simulink model "base_for_gendata"  (R2025a)
settings: Solver=VariableStepAuto  StartTime=0.0  StopTime=inf  RelTol=1e-3
undefined symbols (not defined in the file): Sim3dSensor
libraries: aerolibsim3d x2, sim3dcameralib x1, sl3dlib x1, sim3dphyssensorlib x1, sim3dlib x1, visionsinks x1
settings Model: Creator=Алексей  LastModifiedBy=Алексей

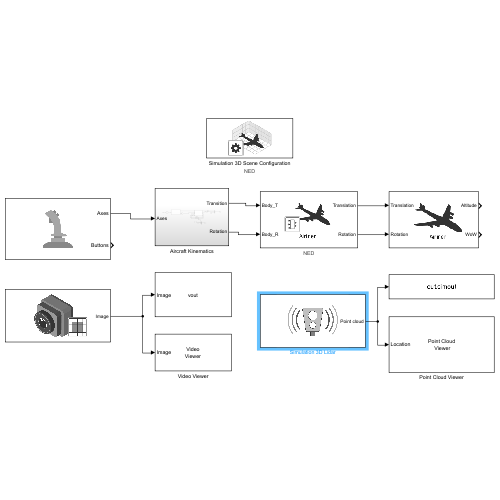
[thumbnail: Simulink's stored preview of the top-level diagram]
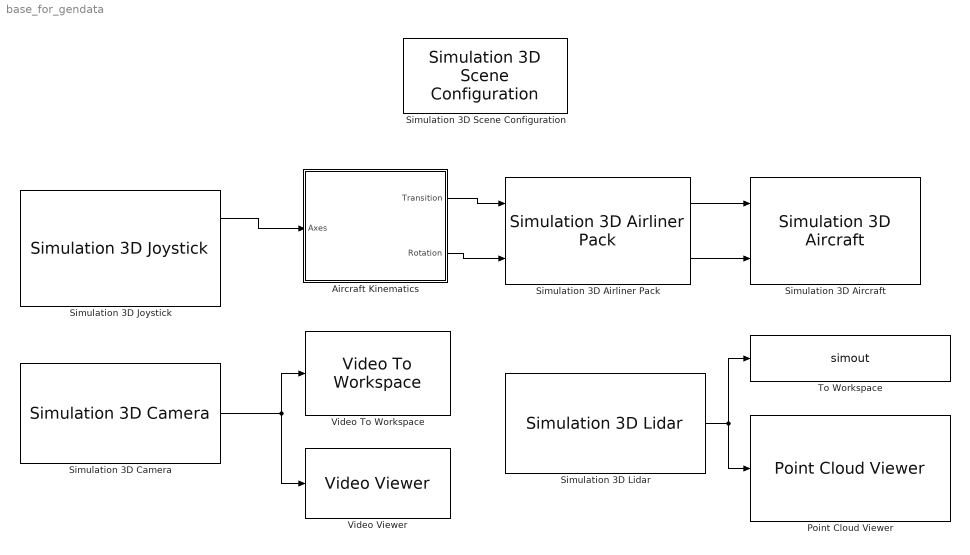
== system base_for_gendata ==
  Aircraft Kinematics : Subsystem
  Point Cloud Viewer : PointCloudViewer  FigPos=[2599 988 1022 472]  FigSettingsValue=[-1 138.910766601562 -120.239807128906 120.152908325195 -3.03508996963501 1 1]
  Simulation 3D Aircraft : aerolibsim3d/Simulation 3D Aircraft  Priority=-1  Mesh=Airliner  MeshPath=/MathWorksAerospaceContent/Vehicles/Aircraft/Custom/Mesh/SK_HL20.SK_HL20  MeshPathAT=/MathWorksAerospaceContent/Vehicles/Aircraft/AirTransport/Mesh/SK_AirTransport.SK_AirTransport  MeshPathGA=/MathWorksAerospaceContent/Vehicles/Aircraft/GeneralAviation/Mesh/SK_GeneralAviation.SK_GeneralAviation  AircraftColor=Red  ActorName=SimulinkVehicle1  Translation=repmat([0, 0, -3.030] + [0, 0, -0.01], 12, 1)  Rotation=repmat([0, -0.00021, 0], 12, 1)  ScaleInputPort=Dialog  Scale=[1 1 1]  InitialScale=[1 1 1]  IsGHSensorEnabled=on  AreGHRaysVisible=off  IsOutputReshapeEnabled=off  GHRayLength=1524  GHBodyOffset=0.90  GHFrontTireRadius=0.21  GHLeftTireRadius=0.21  GHRightTireRadius=0.21  WoWSensorTolerance=0.05  LightsConfig=Automatic lights  LandingLightIntensity=300000  LandingLightConeAngle=15  CustomLeftLandingLightLocation=[0 0 0]  CustomLeftLandingLightOrientation=[0 0 0]  CustomRightLandingLightLocation=[0 0 0]  CustomRightLandingLightOrientation=[0 0 0]  TaxiLightIntensity=150000  TaxiLightConeAngle=36  CustomTaxiLightLocation=[0 0 0]  CustomTaxiLightOrientation=[0 0 0]  NavLightIntensity=500  PositionLightIntensity=500  StrobeLightIntensity=5000  WingtipStrobePeriod=1.5  WingtipStrobePulseWidth=6  TailStrobePeriod=1.5  TailStrobePulseWidth=6  BeaconLightIntensity=4000  BeaconPeriod=1.5  BeaconPulseWidth=10  SampleTime=-1  ActorType=SimulinkVehicle  ID=1  aMode=0  ActorTag=SimulinkVehicle1
  Simulation 3D Airliner Pack : aerolibsim3d/Simulation 3D Airliner Pack  Left_Engine_R=off  Right_Engine_R=off  Rudder_R=off  Elevator_R=off  Left_Aileron_R=off  Right_Aileron_R=off  Flaps_R=off  Nose_Wheel_Strut_R=off  Nose_Wheel_R=off  Left_Wheel_R=off  Right_Wheel_R=off  GeoRadioButton=NED
      settings: AttributesFormatString=NED
  Simulation 3D Camera : sim3dcameralib/Simulation 3D Camera  Priority=1  sensorTag=Sim3dSensor�  sensorId=1  sensorName=Sim3dSensor�  vehTagList={'Scene Origin';'SimulinkVehicle1'}  vehTag=SimulinkVehicle1  CoordinateSystem=Default  mountLoc=Nose  offsetFlag=on  tmountOffset=[0, 0, 0]  extTmount=off  rmountOffset=[0, 0, 0]  extRmount=off  FocalLength=[1109, 1109]  OpticalCenter=[640, 360]  ImageSize=[720, 1280]  RadialDistortion=[0, 0]  TangentialDistortion=[0, 0]  SensorSkew=0  VisualizeFieldOfView=off  FieldOfViewRange=61  DepthOutportEnabled=off  SemanticOutportEnabled=off  TransformOutportEnabled=off  SampleTime=0.1  mountPoint=[12.22 0 -0.26]  mountOrientation=[0 0 0]  aMode=5  ID=1
      settings: LibrarySourceBlock=sl3dlib/Simulation 3D/Sensors/Simulation 3D Camera
  Simulation 3D Joystick : sl3dlib/Simulation 3D/Hardware Interface/Simulation 3D Joystick  joyid=1  adjustports=on  forcefeed=off
  Simulation 3D Lidar : sim3dphyssensorlib/Simulation 3D Lidar  Priority=1  sensorTag=Sim3dSensor�  sensorId=2  sensorName=Sim3dSensor�  vehTagList={'Scene Origin';'SimulinkVehicle1'}  vehTag=SimulinkVehicle1  CoordinateSystem=Default  mountLoc=Nose  offsetFlag=off  tmountOffset=[0, 0, 0]  rmountOffset=[0, 0, 0]  DetectionRange=200  RangeResolution=0.002  VerticalFOV=90  VerticalResolution=1.25  HorizontalFOV=120  HorizontalResolution=0.16  DistanceOutportEnabled=off  ReflectivityOutportEnabled=off  SemanticOutportEnabled=off  TransformOutportEnabled=off  SampleTime=0.1  mountPoint=[12.22 0 -0.26]  mountOrientation=[0 0 0]  aMode=5  ID=2
      settings: LibrarySourceBlock=sl3dlib/Simulation 3D/Sensors/Simulation 3D Lidar
  Simulation 3D Scene Configuration : sim3dlib/Simulation 3D Scene Configuration  Priority=0  ProjectFormat=Default Scenes  SceneDesc=Airport  ProjectName=C:\Program Files\MATLAB\R2025a\toolbox\shared\sim3d_projects\automotive_project_windows\UE\WindowsNoEditor\VehicleSimulation.exe  ScenePath=/Game/Maps/HwStrght  EnableOpenDRIVE=off  vehTagList={'Custom';'Scene Origin';'SimulinkVehicle1'}  vehTag=SimulinkVehicle1  AttachedCameraRelativeTranslation=[0 0 0]  FreeCameraDefaultInitialTranslation=[-6, 0, 2]  AttachedCameraRelativeRotation=[0 0 0]  FreeCameraDefaultInitialRotation=[0, -15, 0]  ViewpointName=Custom  FreeCameraInitialTranslation=[-6, 0, 2]  ViewpointTranslation=[0 0 0]  FreeCameraInitialRotation=[0, -15, 0]  ViewpointRotation=[0 0 0]  OpVisEn=off  Ts=.02  EnableWindow=on  EnableRemoteAccess=off  EnableWeather=off  SunAzimuth=90  SunAltitude=40.0  EnableGeospatialSun=off  Latitude=0  Longitude=0  Date=2023-01-01  Time=10:30:00  GeoTimeZone=-5.0  SunDaylightSaving=off  wind=1  clouds=10  EnableVolumetricClouds=off  CloudCoverage=0  CloudAltitude=6  fog=0  rain=0  RaindropsEffect=off  SnowDensity=0  EnableGeospatial=off  TilesetSource=Earth terrain  UseTrueOrigin=off  OriginHeight=200  OriginLatitude=40.744652  OriginLongitude=-73.988864  MapStyle=Aerial  AdditionalAssetIDs=[]  UseAdvancedSunSky=off  SolarTime=11  TimeZone=-5  Day=21  Month=9  Year=2022  UseDaylightSavingTime=on  DSTStartDay=10  DSTStartMonth=3  DSTEndDay=3  DSTEndMonth=11  DSTSwitchHour=2  sensorTag=MainCamera1  sensorId=1  sensorName=MainCamera1  mountLoc=Origin  offsetFlag=off  tmountOffset=[0, 0, 0]  rmountOffset=[0, 0, 0]  HorizontalResolution=1280  VerticalResolution=720  HorizontalFOV=60  mountPoint=[0 0 0]  mountOrientation=[0 0 0]  aMode=0  ID=1  GeoTrigger=Inactive  ViewNameList={'Custom'}  ViewTranslationList={'[-6 0 2]'}  ViewRotationList={'[0 -15 0]'}
      settings: AttributesFormatString=NED  LibrarySourceBlock=aerolibsim3d/Simulation 3D Scene Configuration
  To Workspace : ToWorkspace  VariableName=simout  SaveFormat=Timeseries  SampleTime=-1
  Video To Workspace : visionsinks/Video To Workspace  VariableName=vout  NumInputs=1  DataLimit=inf  DecimationFactor=1  LogFi=off  InPortLabels=R|G|B
  Video Viewer : VideoViewer  FigPos=[3074 549 1022 445]
  wires:
  Simulation 3D Airliner Pack/1 -> Simulation 3D Aircraft/1
  Simulation 3D Airliner Pack/2 -> Simulation 3D Aircraft/2
  Simulation 3D Joystick/1 -> Aircraft Kinematics/1(Axes)
  Aircraft Kinematics/1(Transition) -> Simulation 3D Airliner Pack/1
  Aircraft Kinematics/2(Rotation) -> Simulation 3D Airliner Pack/2
  Simulation 3D Camera/1 -> Video Viewer/1, Video To Workspace/1
  Simulation 3D Lidar/1 -> Point Cloud Viewer/1, To Workspace/1

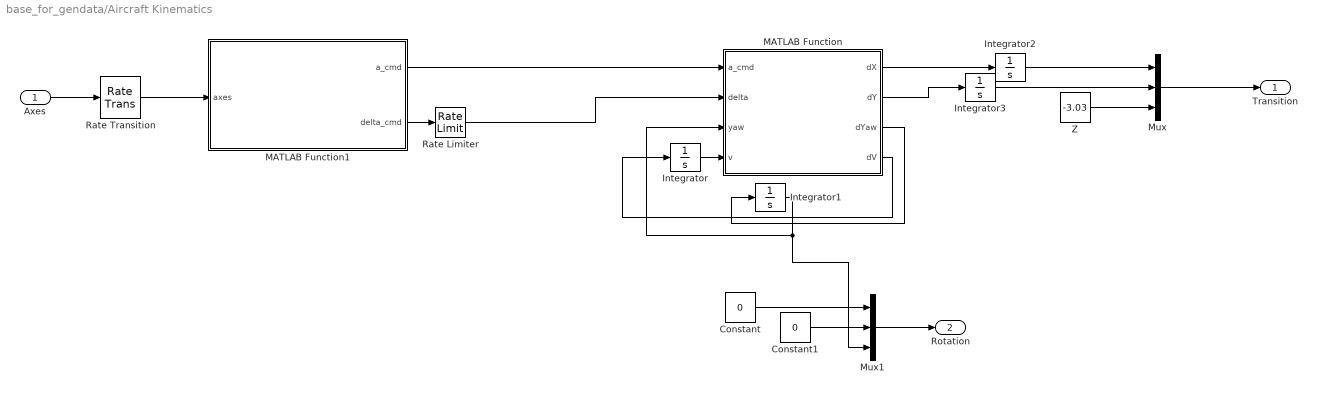
== system base_for_gendata/Aircraft Kinematics ==
  Axes : Inport
  Constant : Constant  Value=0
  Constant1 : Constant  Value=0
  Integrator : Integrator
  Integrator1 : Integrator
  Integrator2 : Integrator  InitialCondition=5500
  Integrator3 : Integrator
  MATLAB Function : MATLAB Function  TreatAsAtomicUnit=on
  MATLAB Function1 : MATLAB Function  TreatAsAtomicUnit=on
  Mux : Mux  Inputs=3
  Mux1 : Mux  Inputs=3
  Rate Limiter : RateLimiter  RisingSlewLimit=0.5  FallingSlewLimit=-0.5  SampleTimeMode=inherited
  Rate Transition : RateTransition
  Z : Constant  Value=-3.03
  Transition : Outport
  Rotation : Outport  Port=2
  wires:
  MATLAB Function1/2(delta_cmd) -> Rate Limiter/1
  Rate Limiter/1 -> MATLAB Function/2(delta)
  Rate Transition/1 -> MATLAB Function1/1(axes)
  Mux1/1 -> Rotation/1
  MATLAB Function/1(dX) -> Integrator2/1
  Constant1/1 -> Mux1/2
  Integrator3/1 -> Mux/2
  MATLAB Function/3(dYaw) -> Integrator1/1
  Mux/1 -> Transition/1
  MATLAB Function1/1(a_cmd) -> MATLAB Function/1(a_cmd)
  MATLAB Function/4(dV) -> Integrator/1
  MATLAB Function/2(dY) -> Integrator3/1
  Constant/1 -> Mux1/1
  Integrator2/1 -> Mux/1
  Integrator/1 -> MATLAB Function/4(v)
  Integrator1/1 -> Mux1/3, MATLAB Function/3(yaw)
  Z/1 -> Mux/3
  Axes/1 -> Rate Transition/1

== matlab function base_for_gendata/Aircraft Kinematics/MATLAB Function1 ==
  data: axes input; a_cmd output; delta_cmd output
function [a_cmd, delta_cmd] = joystick_processor(axes)
    raw_steer = axes(1);
    
    % ИНВЕРСИЯ ТРИГГЕРОВ: 
    % Теперь правый триггер (который давал минус) станет положительным (газ),
    % а левый (который давал плюс) станет отрицательным (тормоз).
    raw_throttle = -axes(3); 
    
    % Мертвая зона для руля
    if abs(raw_steer) < 0.1
        raw_steer = 0;
    end
    
    % Угол поворота (максимум 0.5 рад)
    delta_cmd = raw_steer * 0.5;
    
    % Газ и тормоз
    if raw_throttle > 0.1
        a_cmd = raw_throttle * 2.0;  % Теперь это правый триггер (Газ)
    elseif raw_throttle < -0.1
        a_cmd = raw_throttle * 3.0;  % Теперь это левый триггер (Тормоз)
    else
        a_cmd = 0; 
    end
end

== matlab function base_for_gendata/Aircraft Kinematics/MATLAB Function ==
  data: a_cmd input; dX output; dY output; delta input; yaw input; v input; dYaw output; dV output
function [dX, dY, dYaw, dV] = vehicle_kinematics(a_cmd, delta, yaw, v)
    % L - база шасси (примерно 15 метров)
    L = 15; 
    
    % Коэффициент сопротивления (имитация трения качения и сопротивления воздуха)
    % Чем больше число, тем быстрее самолет останавливается
    drag = 0.1; 
    
    % Внутри функции vehicle_kinematics
    max_delta_at_speed = 0.6 * (1 - min(v/20, 0.8)); % Пример: на скорости 20 м/с угол падает до 20% от максимума
    delta = max(min(delta, max_delta_at_speed), -max_delta_at_speed);

    % 1. Динамика по скорости (ускорение минус сопротивление)
    dV = a_cmd - drag * v;
    
    % Ограничение: самолет не может ехать назад (если только это не pushback)
    if v <= 0 && dV < 0
        dV = 0;
    end
    
    % Ограничение максимальной скорости (например, 15 м/с)
    if v > 30 && dV > 0
        dV = 0;
    end
    
    % 2. Кинематика (Bicycle Model)
    dX = v * cos(yaw);
    dY = v * sin(yaw);
    
    % Угловая скорость зависит от скорости и угла поворота стойки
    dYaw = (v / L) * tan(delta);
end
